simulink model "UAV_Sim"  (R2025b)
settings: Solver=VariableStepAuto  StartTime=0.0  StopTime=10  RelTol=1e-3
undefined symbols (not defined in the file): quad_m, W
libraries: aerolibanimutils x1, uavutilslib x1
settings Model: Creator=Aorus PC  LastModifiedBy=David
settings OptimizationCC: ReuseModelBlockBuffer=off
settings DebuggingCC: UnderspecifiedInitializationDetection=Classic  MergeDetectMultiDrivingBlocksExec=none
settings ModelReferenceCC: PropagateSignalLabelsOutOfModel=off
settings RTWCC: GPUComputeCapability=3.5

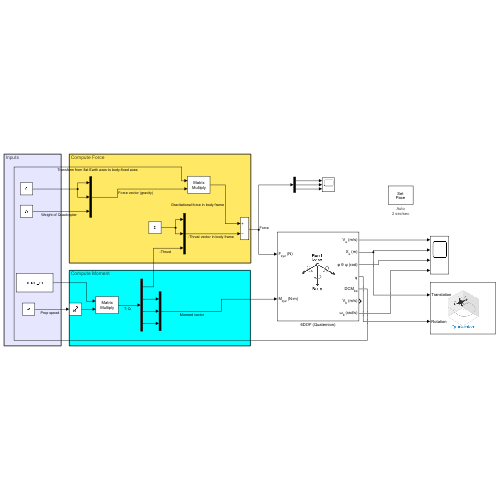
[thumbnail: Simulink's stored preview of the top-level diagram]
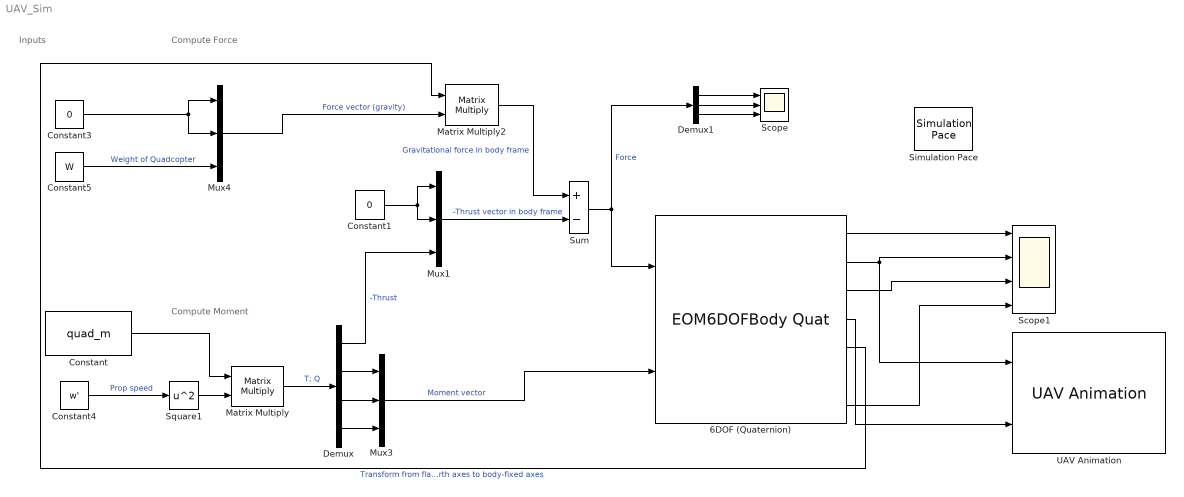
== system UAV_Sim ==
  note: Compute Moment
  note: Compute Force
  note: Inputs
  6DOF (Quaternion) : EOM6DOFBodyQuat
  Constant : Constant  Value=quad_m
  Constant1 : Constant  Value=0
  Constant3 : Constant  Value=0
  Constant4 : Constant  Value=w'
  Constant5 : Constant  Value=W
  Demux : Demux
  Demux1 : Demux  Outputs=3
  Matrix Multiply : Product  Multiplication=Matrix(*)
  Matrix Multiply2 : Product  Multiplication=Matrix(*)
  Mux1 : Mux  Inputs=3
  Mux3 : Mux  Inputs=3
  Mux4 : Mux  Inputs=3
  Scope : Scope  NumInputPorts=3
      settings: ActiveDisplayYMinimum=-1  ActiveDisplayYMaximum=1
  Scope1 : Scope  NumInputPorts=4
      settings: ActiveDisplayYMinimum=-1  ActiveDisplayYMaximum=1
  Simulation Pace : aerolibanimutils/Simulation Pace  SimulationPace=2  SleepMode=Auto  OutputPaceError=off  SampleTime=1/30
  Square1 : Math  Operator=square
  Sum : Sum  Inputs=+-
  UAV Animation : uavutilslib/UAV Animation  NumUAV=1  DynamicUAVConfig=off  UAVType=Multirotor  UAVSize=4  UAVColor=[1 0 0]  UAVTrajectoryAlpha=1  InertialZDirection=Down  RotationFormat=Quaternion  DrawMarkers=off  SampleTime=-1
  wires:
  Constant/1 -> Matrix Multiply/1
  Matrix Multiply/1 -> Demux/1  "T; Q"
  Demux/2 -> Mux3/1
  Demux/3 -> Mux3/2
  Demux/4 -> Mux3/3
  Mux3/1 -> 6DOF (Quaternion)/2  "Moment vector"
  Constant3/1 -> Mux4/1, Mux4/2
  Constant5/1 -> Mux4/3  "Weight of Quadcopter"
  Constant1/1 -> Mux1/1, Mux1/2
  Square1/1 -> Matrix Multiply/2
  Demux/1 -> Mux1/3  "-Thrust"
  Constant4/1 -> Square1/1  "Prop speed"
  Demux1/2 -> Scope/2
  Demux1/1 -> Scope/1
  Demux1/3 -> Scope/3
  Sum/1 -> Demux1/1, 6DOF (Quaternion)/1  "Force"
  6DOF (Quaternion)/2 -> UAV Animation/1, Scope1/2
  Mux4/1 -> Matrix Multiply2/2  "Force vector (gravity)"
  Matrix Multiply2/1 -> Sum/1  "Gravitational force in body frame"
  Mux1/1 -> Sum/2  "-Thrust vector in body frame"
  6DOF (Quaternion)/4 -> UAV Animation/2
  6DOF (Quaternion)/5 -> Matrix Multiply2/1  "Transform from flat Earth axes to body-fixed axes"
  6DOF (Quaternion)/1 -> Scope1/1
  6DOF (Quaternion)/7 -> Scope1/4
  6DOF (Quaternion)/3 -> Scope1/3
